simulink model "CompleteSystem"  (R2026a)
settings: Solver=VariableStepAuto
InitFcn:
  | addpath('C:/Users/lucas/MATLAB/Projects/TVC^2/Multibody/cad_export');
  | run('C:/Users/lucas/MATLAB/Projects/TVC^2/Multibody/cad_export/FullAssembly_DataFile.m');
  | addpath('C:/Users/lucas/MATLAB/Projects/TVC^2/Params');
  | run('C:/Users/lucas/MATLAB/Projects/TVC^2/Params/RocketParameter.m');
  | run('C:/Users/lucas/MATLAB/Projects/TVC^2/Params/InitialConditions.m');
libraries: rocket_multibody_lib x1
settings Model: Creator=lucas  LastModifiedBy=lucas

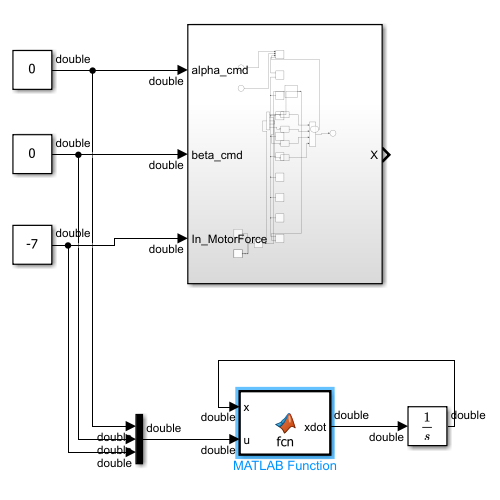
[thumbnail: Simulink's stored preview of the top-level diagram]
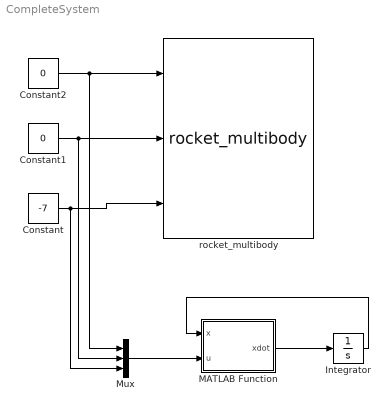
== system CompleteSystem ==
  Constant : Constant  Value=-7
  Constant1 : Constant  Value=0
  Constant2 : Constant  Value=0
  Integrator : Integrator
  MATLAB Function : MATLAB Function  TreatAsAtomicUnit=on
  Mux : Mux  Inputs=3
  rocket_multibody : rocket_multibody_lib/rocket_multibody  SystemSampleTime=-1  VariantActivationTime=update diagram  EmptyChoice=off  PassThrough=off  PassThroughVariantControl=(default)  EmptyChoiceVariantControl=(default)  AllowFlexibleInterface=on  Latency=0  AutoFrameSizeCalculation=off
  wires:
  Constant/1 -> Mux/3, rocket_multibody/3
  Constant1/1 -> Mux/2, rocket_multibody/2
  Constant2/1 -> Mux/1, rocket_multibody/1
  Mux/1 -> MATLAB Function/2(u)
  MATLAB Function/1(xdot) -> Integrator/1
  Integrator/1 -> MATLAB Function/1(x)

== matlab function CompleteSystem/MATLAB Function ==
  data: x input size=[16 1]; u input; xdot output size=[16 1]; P parameter
function xdot = fcn(x,u,P)

xdot = zeros(16,1);

temp = Dynamics(x,u,P);

for i = 1:16
    xdot(i) = temp(i);
end

end
